simulink model "HPP"  (R2026a)
settings: Solver=ode1  StopTime=p.sim.Tstop  FixedStep=HPP_Tnet
model workspace (MAT data in the model file):
  HPP_Tnet = 0.001
  HPP_Ts = 0.001
  HPP_delays = 1
  HPP_f0 = 50
  HPP_network = 1
  HPP_simscape = 1
  buildInfo : object (value not decoded)
undefined symbols (not defined in the file): p
libraries: ee_lib x57, nesl_utility x29, fl_lib x6
(part 3 of 5)

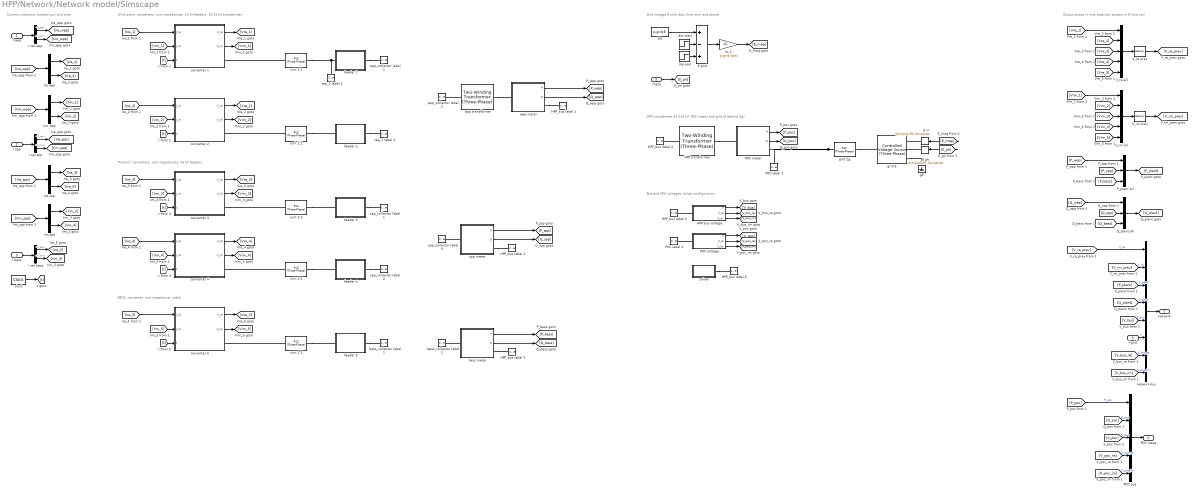
== system HPP/Network/Network model/Simscape ==
  note: Current injections (system pu) and time
  note: Wind plant: converters, unit impedances, 10 kV feeders, 10-33 kV transformer
  note: PV plant: converters, unit impedances, 33 kV feeders
  note: BESS: converter, unit impedance, cable
  note: Grid voltage E with dips (line rms) and phase
  note: HPP transformer 33-132 kV, POC meter and grid (E behind Zg)
  note: Bus and POC voltages, solver configuration
  note: Output buses (V one step old, powers in W and var)
  I wpp : Inport
  I spp : Inport  Port=2
  I bess : Inport  Port=3
  f grid : Inport  Port=4
  theta : Inport  Port=5
  E grid : Sum  Inputs=+-+
  E in : nesl_utility/Simulink-PS Converter  PhysicalDomain=network_engine_domain  SubClassName=ps_input  LeftPortType=input  RightPortType=output  PseudoPeriodic=off  Frequencies=[]  NoiseDistribution=none  NoiseParameters=[]  Unit=V  AffineConversion=off  FilteringAndDerivatives=provide  SimscapeFilterOrder=1  InputFilterTimeConstant=0.001  UdotUserProvided=0
  E ph : nesl_utility/Simulink-PS Converter  PhysicalDomain=network_engine_domain  SubClassName=ps_input  LeftPortType=input  RightPortType=output  PseudoPeriodic=off  Frequencies=[]  NoiseDistribution=none  NoiseParameters=[]  Unit=rad  AffineConversion=off  FilteringAndDerivatives=provide  SimscapeFilterOrder=1  InputFilterTimeConstant=0.001  UdotUserProvided=0
  E0 : Constant  Value=p.grid.E
  HPP bus voltage : Subsystem
  HPP transformer : ee_lib/Passive/Transformers/Two-Winding Transformer (Three-Phase)  SRated=p.net.main.S A*V  FRated=HPP_f0 Hz  Winding1Connection=ee.enum.windingconnection.Yg  VRated1=p.net.Vhpp V  Winding2Connection=ee.enum.windingconnection.Yg  VRated2=p.grid.Vpoc V  CoreType=ee.enum.coretype.threelimb  pu_Rw1=(p.net.main.uk/sqrt(1+p.net.main.XR^2))/2  pu_Rw2=(p.net.main.uk/sqrt(1+p.net.main.XR^2))/2  leakage_reactance_option=ee.enum.transformer_leakage.include  pu_Xl1=(p.net.main.uk/sqrt(1+p.net.main.XR^2))*p.net.main.XR/2  pu_Xl2=(p.net.main.uk/sqrt(1+p.net.main.XR^2))*p.net.main.XR/2  magnetizing_resistance_option=ee.enum.transformer_magnetizingResistance.include  pu_Rm=p.net.main.Rm  magnetizing_reactance_option=ee.enum.transformer_magnetizingReactance.include  saturation_option=ee.enum.transformer_saturation.exclude  pu_Xm=p.net.main.Xm  current_data=[0, .002, 1, 2]  magnetic_flux_data=[0, 1.2, 1.5, 1.51]  pu_X0=0.5  i1_specify=off  i1_priority=None  i1=[0, 0, 0] A  i1_nominal_specify=off  i1_nominal_value=1  i1_nominal_unit=A  i2_specify=off  i2_priority=None  i2=[0, 0, 0] A  i2_nominal_specify=off  i2_nominal_value=1  i2_nominal_unit=A  phi_specify=off  phi_priority=None  phi=[0, 0, 0]  phi_nominal_specify=off  phi_nominal_value=1  phi_nominal_unit=1
  HPP_bus label {1..6} (6 alike) : ConnectionLabel  Label=HPP_bus
  I sel bess : BusSelector  OutputSignals=I_re,I_im
  I sel spp : BusSelector  OutputSignals=I_re,I_im
  I sel wpp : BusSelector  OutputSignals=I_re,I_im
  Iim spp : Demux  Outputs=2
  Iim wpp : Demux  Outputs=2
  Ire spp : Demux  Outputs=2
  Ire wpp : Demux  Outputs=2
  POC bus : BusCreator  Inputs=5
  POC label 1 : ConnectionLabel  Label=POC
  POC label 2 : ConnectionLabel  Label=POC
  POC meter : Subsystem
  POC voltage : Subsystem
  P_plant all : Mux  Inputs=3
  Q_plant all : Mux  Inputs=3
  V_im all : Mux  Inputs=5
  V_im prev : Memory  InitialCondition=zeros(5,1)
  V_re all : Mux  Inputs=5
  V_re prev : Memory  InitialCondition=ones(5,1)
  bess meter : Subsystem
  bess_collector label 1 : ConnectionLabel  Label=bess_collector
  bess_collector label 2 : ConnectionLabel  Label=bess_collector
  clock : DigitalClock  SampleTime=HPP_Ts
  converter 1 : Subsystem
  converter 2 : Subsystem
  converter 3 : Subsystem
  converter 4 : Subsystem
  converter 5 : Subsystem
  dip end : Step  Time=p.grid.dip.t0 + p.grid.dip.dur  FinalValue=p.grid.dip.depth  SampleTime=0
  dip start : Step  Time=p.grid.dip.t0  FinalValue=p.grid.dip.depth  SampleTime=0
  feeder 1 : Subsystem
  feeder 2 : Subsystem
  feeder 3 : Subsystem
  feeder 4 : Subsystem
  feeder 5 : Subsystem
  gE : fl_lib/Electrical/Electrical Elements/Electrical Reference
  grid E : ee_lib/Sources/Controlled Voltage Source (Three-Phase)  input_option=ee.enum.inputType.singleFreqAC  FRated=HPP_f0 Hz
  grid Zg : ee_lib/Passive/RLC Assemblies/RLC (Three-Phase)  port_option=ee.enum.threePhasePort.composite  component_structure=ee.enum.rlc.structure.SeriesRL  R=(p.grid.Vpoc^2/(p.grid.SCR*p.grid.Pmax_poc))/sqrt(1+p.grid.XR^2) Ohm  L=(p.grid.Vpoc^2/(p.grid.SCR*p.grid.Pmax_poc))*p.grid.XR/sqrt(1+p.grid.XR^2)/(2*pi*p.grid.f0) H  C=1e-6 F  R_parasitic=0 Ohm  G_parasitic=0 1/Ohm  IL_specify=off  IL_priority=High  IL=[0, 0, 0] A  IL_nominal_specify=off  IL_nominal_value=1  IL_nominal_unit=A  VC_specify=off  VC_priority=High  VC=[0, 0, 0] V  VC_nominal_specify=off  VC_nominal_value=1  VC_nominal_unit=V
  network bus : BusCreator  Inputs=8
  solver : Subsystem  Description=Simscape solver, chosen per run by HPP_simscape (p.net.simscapeMode): Phasor (1, frequency-and-time mode, step p.sim.Ts) or EMT (2, time mode, step p.net.emtTs). See simscapeMode.  Variant=on
  spp meter : Subsystem
  spp_collector label 1 : ConnectionLabel  Label=spp_collector
  spp_collector label 2 : ConnectionLabel  Label=spp_collector
  spp_collector label 3 : ConnectionLabel  Label=spp_collector
  tap_1 label 1 : ConnectionLabel  Label=tap_1
  tap_1 label 2 : ConnectionLabel  Label=tap_1
  to V : Gain  Gain=p.grid.Vpoc
  unit Z 1 : ee_lib/Passive/RLC Assemblies/RLC (Three-Phase)  port_option=ee.enum.threePhasePort.composite  component_structure=ee.enum.rlc.structure.SeriesRL  R=(p.net.wt.unit.uk*p.net.wt.Vcol^2/(p.net.wt.unit.S*p.wt.nAgg))/sqrt(1+p.net.wt.unit.XR^2) Ohm  L=(p.net.wt.unit.uk*p.net.wt.Vcol^2/(p.net.wt.unit.S*p.wt.nAgg))*p.net.wt.unit.XR/sqrt(1+p.net.wt.unit.XR^2)/(2*pi*p.grid.f0) H  C=1e-6 F  R_parasitic=0 Ohm  G_parasitic=0 1/Ohm  IL_specify=off  IL_priority=High  IL=[0, 0, 0] A  IL_nominal_specify=off  IL_nominal_value=1  IL_nominal_unit=A  VC_specify=off  VC_priority=High  VC=[0, 0, 0] V  VC_nominal_specify=off  VC_nominal_value=1  VC_nominal_unit=V
  unit Z 2 : ee_lib/Passive/RLC Assemblies/RLC (Three-Phase)  port_option=ee.enum.threePhasePort.composite  component_structure=ee.enum.rlc.structure.SeriesRL  R=(p.net.wt.unit.uk*p.net.wt.Vcol^2/(p.net.wt.unit.S*p.wt.nAgg))/sqrt(1+p.net.wt.unit.XR^2) Ohm  L=(p.net.wt.unit.uk*p.net.wt.Vcol^2/(p.net.wt.unit.S*p.wt.nAgg))*p.net.wt.unit.XR/sqrt(1+p.net.wt.unit.XR^2)/(2*pi*p.grid.f0) H  C=1e-6 F  R_parasitic=0 Ohm  G_parasitic=0 1/Ohm  IL_specify=off  IL_priority=High  IL=[0, 0, 0] A  IL_nominal_specify=off  IL_nominal_value=1  IL_nominal_unit=A  VC_specify=off  VC_priority=High  VC=[0, 0, 0] V  VC_nominal_specify=off  VC_nominal_value=1  VC_nominal_unit=V
  unit Z 3 : ee_lib/Passive/RLC Assemblies/RLC (Three-Phase)  port_option=ee.enum.threePhasePort.composite  component_structure=ee.enum.rlc.structure.SeriesRL  R=(p.net.pv.unit.uk*p.net.pv.Vcol^2/(p.net.pv.unit.S*p.pv.nAgg))/sqrt(1+p.net.pv.unit.XR^2) Ohm  L=(p.net.pv.unit.uk*p.net.pv.Vcol^2/(p.net.pv.unit.S*p.pv.nAgg))*p.net.pv.unit.XR/sqrt(1+p.net.pv.unit.XR^2)/(2*pi*p.grid.f0) H  C=1e-6 F  R_parasitic=0 Ohm  G_parasitic=0 1/Ohm  IL_specify=off  IL_priority=High  IL=[0, 0, 0] A  IL_nominal_specify=off  IL_nominal_value=1  IL_nominal_unit=A  VC_specify=off  VC_priority=High  VC=[0, 0, 0] V  VC_nominal_specify=off  VC_nominal_value=1  VC_nominal_unit=V
  unit Z 4 : ee_lib/Passive/RLC Assemblies/RLC (Three-Phase)  port_option=ee.enum.threePhasePort.composite  component_structure=ee.enum.rlc.structure.SeriesRL  R=(p.net.pv.unit.uk*p.net.pv.Vcol^2/(p.net.pv.unit.S*p.pv.nAgg))/sqrt(1+p.net.pv.unit.XR^2) Ohm  L=(p.net.pv.unit.uk*p.net.pv.Vcol^2/(p.net.pv.unit.S*p.pv.nAgg))*p.net.pv.unit.XR/sqrt(1+p.net.pv.unit.XR^2)/(2*pi*p.grid.f0) H  C=1e-6 F  R_parasitic=0 Ohm  G_parasitic=0 1/Ohm  IL_specify=off  IL_priority=High  IL=[0, 0, 0] A  IL_nominal_specify=off  IL_nominal_value=1  IL_nominal_unit=A  VC_specify=off  VC_priority=High  VC=[0, 0, 0] V  VC_nominal_specify=off  VC_nominal_value=1  VC_nominal_unit=V
  unit Z 5 : ee_lib/Passive/RLC Assemblies/RLC (Three-Phase)  port_option=ee.enum.threePhasePort.composite  component_structure=ee.enum.rlc.structure.SeriesRL  R=(p.net.bess.unit.uk*p.net.bess.Vcol^2/(p.net.bess.unit.S*p.bess.nAgg))/sqrt(1+p.net.bess.unit.XR^2) Ohm  L=(p.net.bess.unit.uk*p.net.bess.Vcol^2/(p.net.bess.unit.S*p.bess.nAgg))*p.net.bess.unit.XR/sqrt(1+p.net.bess.unit.XR^2)/(2*pi*p.grid.f0) H  C=1e-6 F  R_parasitic=0 Ohm  G_parasitic=0 1/Ohm  IL_specify=off  IL_priority=High  IL=[0, 0, 0] A  IL_nominal_specify=off  IL_nominal_value=1  IL_nominal_unit=A  VC_specify=off  VC_priority=High  VC=[0, 0, 0] V  VC_nominal_specify=off  VC_nominal_value=1  VC_nominal_unit=V
  wpp meter : Subsystem
  wpp transformer : ee_lib/Passive/Transformers/Two-Winding Transformer (Three-Phase)  SRated=p.net.wt.plant.S A*V  FRated=HPP_f0 Hz  Winding1Connection=ee.enum.windingconnection.Yg  VRated1=p.net.wt.Vcol V  Winding2Connection=ee.enum.windingconnection.Yg  VRated2=p.net.Vhpp V  CoreType=ee.enum.coretype.threelimb  pu_Rw1=(p.net.wt.plant.uk/sqrt(1+p.net.wt.plant.XR^2))/2  pu_Rw2=(p.net.wt.plant.uk/sqrt(1+p.net.wt.plant.XR^2))/2  leakage_reactance_option=ee.enum.transformer_leakage.include  pu_Xl1=(p.net.wt.plant.uk/sqrt(1+p.net.wt.plant.XR^2))*p.net.wt.plant.XR/2  pu_Xl2=(p.net.wt.plant.uk/sqrt(1+p.net.wt.plant.XR^2))*p.net.wt.plant.XR/2  magnetizing_resistance_option=ee.enum.transformer_magnetizingResistance.include  pu_Rm=p.net.wt.plant.Rm  magnetizing_reactance_option=ee.enum.transformer_magnetizingReactance.include  saturation_option=ee.enum.transformer_saturation.exclude  pu_Xm=p.net.wt.plant.Xm  current_data=[0, .002, 1, 2]  magnetic_flux_data=[0, 1.2, 1.5, 1.51]  pu_X0=0.5  i1_specify=off  i1_priority=None  i1=[0, 0, 0] A  i1_nominal_specify=off  i1_nominal_value=1  i1_nominal_unit=A  i2_specify=off  i2_priority=None  i2=[0, 0, 0] A  i2_nominal_specify=off  i2_nominal_value=1  i2_nominal_unit=A  phi_specify=off  phi_priority=None  phi=[0, 0, 0]  phi_nominal_specify=off  phi_nominal_value=1  phi_nominal_unit=1
  wpp_collector label 1 : ConnectionLabel  Label=wpp_collector
  wpp_collector label 2 : ConnectionLabel  Label=wpp_collector
  network : Outport
  POC meas : Outport  Port=2
  wires:
  I wpp/1 -> I sel wpp/1
  I sel wpp/2 -> [Iim_wpp]  "<I_im>"
  I sel wpp/1 -> [Ire_wpp]  "<I_re>"
  [Ire_wpp] -> Ire wpp/1
  Ire wpp/2 -> [Ire_2]
  Ire wpp/1 -> [Ire_1]
  [Iim_wpp] -> Iim wpp/1
  Iim wpp/2 -> [Iim_2]
  Iim wpp/1 -> [Iim_1]
  I spp/1 -> I sel spp/1
  I sel spp/2 -> [Iim_spp]  "<I_im>"
  I sel spp/1 -> [Ire_spp]  "<I_re>"
  [Ire_spp] -> Ire spp/1
  Ire spp/2 -> [Ire_4]
  Ire spp/1 -> [Ire_3]
  [Iim_spp] -> Iim spp/1
  Iim spp/2 -> [Iim_4]
  Iim spp/1 -> [Iim_3]
  I bess/1 -> I sel bess/1
  I sel bess/2 -> [Iim_5]  "<I_im>"
  I sel bess/1 -> [Ire_5]  "<I_re>"
  clock/1 -> [t]
  [Ire_1] -> converter 1/1(I_re)
  [Iim_1] -> converter 1/2(I_im)
  [t] -> converter 1/3(t)
  converter 1/2(V_im) -> [Vim_1]
  converter 1/1(V_re) -> [Vre_1]
  [Ire_2] -> converter 2/1(I_re)
  [Iim_2] -> converter 2/2(I_im)
  [t] -> converter 2/3(t)
  converter 2/2(V_im) -> [Vim_2]
  converter 2/1(V_re) -> [Vre_2]
  wpp meter/1(P) -> [P_wpp]
  wpp meter/2(Q) -> [Q_wpp]
  [Ire_3] -> converter 3/1(I_re)
  [Iim_3] -> converter 3/2(I_im)
  [t] -> converter 3/3(t)
  converter 3/2(V_im) -> [Vim_3]
  converter 3/1(V_re) -> [Vre_3]
  [Ire_4] -> converter 4/1(I_re)
  [Iim_4] -> converter 4/2(I_im)
  [t] -> converter 4/3(t)
  converter 4/2(V_im) -> [Vim_4]
  converter 4/1(V_re) -> [Vre_4]
  spp meter/1(P) -> [P_spp]
  spp meter/2(Q) -> [Q_spp]
  [Ire_5] -> converter 5/1(I_re)
  [Iim_5] -> converter 5/2(I_im)
  [t] -> converter 5/3(t)
  converter 5/2(V_im) -> [Vim_5]
  converter 5/1(V_re) -> [Vre_5]
  bess meter/1(P) -> [P_bess]
  bess meter/2(Q) -> [Q_bess]
  E0/1 -> E grid/1
  dip start/1 -> E grid/2
  dip end/1 -> E grid/3
  E grid/1 -> to V/1
  to V/1 -> [E_mag]
  theta/1 -> [E_ph]
  [E_mag] -> E in/1
  [E_ph] -> E ph/1
  POC meter/1(P) -> [P_poc]
  POC meter/2(Q) -> [Q_poc]
  HPP bus voltage/1(V) -> [V_bus]
  HPP bus voltage/2(V_re) -> [V_bus_re]
  HPP bus voltage/3(V_im) -> [V_bus_im]
  POC voltage/1(V) -> [V_poc]
  POC voltage/2(V_re) -> [V_poc_re]
  POC voltage/3(V_im) -> [V_poc_im]
  [Vre_1] -> V_re all/1
  [Vre_2] -> V_re all/2
  [Vre_3] -> V_re all/3
  [Vre_4] -> V_re all/4
  [Vre_5] -> V_re all/5
  V_re all/1 -> V_re prev/1
  V_re prev/1 -> [V_re_prev]
  [Vim_1] -> V_im all/1
  [Vim_2] -> V_im all/2
  [Vim_3] -> V_im all/3
  [Vim_4] -> V_im all/4
  [Vim_5] -> V_im all/5
  V_im all/1 -> V_im prev/1
  V_im prev/1 -> [V_im_prev]
  [P_wpp] -> P_plant all/1
  [P_spp] -> P_plant all/2
  [P_bess] -> P_plant all/3
  P_plant all/1 -> [P_plant]
  [Q_wpp] -> Q_plant all/1
  [Q_spp] -> Q_plant all/2
  [Q_bess] -> Q_plant all/3
  Q_plant all/1 -> [Q_plant]
  [V_re_prev] -> network bus/1  "V_re"
  [V_im_prev] -> network bus/2  "V_im"
  [P_plant] -> network bus/3  "P_plant"
  [Q_plant] -> network bus/4  "Q_plant"
  [V_bus] -> network bus/5  "V_bus"
  f grid/1 -> network bus/6  "f"
  [V_bus_re] -> network bus/7  "V_bus_re"
  [V_bus_im] -> network bus/8  "V_bus_im"
  network bus/1 -> network/1
  [P_poc] -> POC bus/1  "P_poc"
  [Q_poc] -> POC bus/2  "Q_poc"
  [V_poc] -> POC bus/3  "V_poc"
  [V_poc_re] -> POC bus/4  "V_poc_re"
  [V_poc_im] -> POC bus/5  "V_poc_im"
  POC bus/1 -> POC meas/1
  connections:
  converter 1/RConn1 -- unit Z 1/LConn1
  feeder 1/LConn1 -- unit Z 1/RConn1 -- tap_1 label 1/LConn1
  feeder 1/RConn1 -- wpp_collector label 1/LConn1
  converter 2/RConn1 -- unit Z 2/LConn1
  unit Z 2/RConn1 -- feeder 2/LConn1
  feeder 2/RConn1 -- tap_1 label 2/LConn1
  wpp transformer/LConn1 -- wpp_collector label 2/LConn1
  wpp transformer/RConn1 -- wpp meter/LConn1
  wpp meter/RConn1 -- HPP_bus label 1/LConn1
  converter 3/RConn1 -- unit Z 3/LConn1
  unit Z 3/RConn1 -- feeder 3/LConn1
  feeder 3/RConn1 -- spp_collector label 1/LConn1
  converter 4/RConn1 -- unit Z 4/LConn1
  unit Z 4/RConn1 -- feeder 4/LConn1
  feeder 4/RConn1 -- spp_collector label 2/LConn1
  spp meter/LConn1 -- spp_collector label 3/LConn1
  spp meter/RConn1 -- HPP_bus label 2/LConn1
  converter 5/RConn1 -- unit Z 5/LConn1
  unit Z 5/RConn1 -- feeder 5/LConn1
  feeder 5/RConn1 -- bess_collector label 1/LConn1
  bess meter/LConn1 -- bess_collector label 2/LConn1
  bess meter/RConn1 -- HPP_bus label 3/LConn1
  HPP transformer/LConn1 -- HPP_bus label 4/LConn1
  HPP transformer/RConn1 -- POC meter/LConn1
  grid Zg/LConn1 -- POC meter/RConn1 -- POC label 1/LConn1
  grid Zg/RConn1 -- grid E/RConn1
  grid E/LConn3 -- gE/LConn1
  E in/RConn1 -- grid E/LConn1
  E ph/RConn1 -- grid E/LConn2
  HPP bus voltage/LConn1 -- HPP_bus label 5/LConn1
  POC voltage/LConn1 -- POC label 2/LConn1
  solver/RConn1 -- HPP_bus label 6/LConn1

== system HPP/PV plant/P_avail_k link/delay 3 ==
  note: 1) Add Subsystem or Model blocks as valid variant choices.
      | 2) You cannot connect blocks at this level. At simulation, connectivity is automatically
      | determined, based on the active variant and port name matching.
  u : Inport
  Fixed : Subsystem  VariantControl=HPP_delays == 1
  Variable : Subsystem  VariantControl=HPP_delays == 2
  y : Outport

== system HPP/PV plant/P_meas link/delay 3 ==
  note: 1) Add Subsystem or Model blocks as valid variant choices.
      | 2) You cannot connect blocks at this level. At simulation, connectivity is automatically
      | determined, based on the active variant and port name matching.
  u : Inport
  Fixed : Subsystem  VariantControl=HPP_delays == 1
  Variable : Subsystem  VariantControl=HPP_delays == 2
  y : Outport

== system HPP/PV plant/P_set link/delay 1 ==
  note: 1) Add Subsystem or Model blocks as valid variant choices.
      | 2) You cannot connect blocks at this level. At simulation, connectivity is automatically
      | determined, based on the active variant and port name matching.
  u : Inport
  Fixed : Subsystem  VariantControl=HPP_delays == 1
  Variable : Subsystem  VariantControl=HPP_delays == 2
  y : Outport

== system HPP/PV plant/P_set_k link/delay 1 ==
  note: 1) Add Subsystem or Model blocks as valid variant choices.
      | 2) You cannot connect blocks at this level. At simulation, connectivity is automatically
      | determined, based on the active variant and port name matching.
  u : Inport
  Fixed : Subsystem  VariantControl=HPP_delays == 1
  Variable : Subsystem  VariantControl=HPP_delays == 2
  y : Outport

== system HPP/PV plant/Q_meas link/delay 3 ==
  note: 1) Add Subsystem or Model blocks as valid variant choices.
      | 2) You cannot connect blocks at this level. At simulation, connectivity is automatically
      | determined, based on the active variant and port name matching.
  u : Inport
  Fixed : Subsystem  VariantControl=HPP_delays == 1
  Variable : Subsystem  VariantControl=HPP_delays == 2
  y : Outport

== system HPP/PV plant/Q_set link/delay 1 ==
  note: 1) Add Subsystem or Model blocks as valid variant choices.
      | 2) You cannot connect blocks at this level. At simulation, connectivity is automatically
      | determined, based on the active variant and port name matching.
  u : Inport
  Fixed : Subsystem  VariantControl=HPP_delays == 1
  Variable : Subsystem  VariantControl=HPP_delays == 2
  y : Outport

== system HPP/PV plant/Q_set_k link/delay 1 ==
  note: 1) Add Subsystem or Model blocks as valid variant choices.
      | 2) You cannot connect blocks at this level. At simulation, connectivity is automatically
      | determined, based on the active variant and port name matching.
  u : Inport
  Fixed : Subsystem  VariantControl=HPP_delays == 1
  Variable : Subsystem  VariantControl=HPP_delays == 2
  y : Outport

== system HPP/PV plant/V_meas link/delay 2 ==
  note: 1) Add Subsystem or Model blocks as valid variant choices.
      | 2) You cannot connect blocks at this level. At simulation, connectivity is automatically
      | determined, based on the active variant and port name matching.
  u : Inport
  Fixed : Subsystem  VariantControl=HPP_delays == 1
  Variable : Subsystem  VariantControl=HPP_delays == 2
  y : Outport

== system HPP/Wind plant/P_avail_k link/delay 3 ==
  note: 1) Add Subsystem or Model blocks as valid variant choices.
      | 2) You cannot connect blocks at this level. At simulation, connectivity is automatically
      | determined, based on the active variant and port name matching.
  u : Inport
  Fixed : Subsystem  VariantControl=HPP_delays == 1
  Variable : Subsystem  VariantControl=HPP_delays == 2
  y : Outport

== system HPP/Wind plant/P_meas link/delay 3 ==
  note: 1) Add Subsystem or Model blocks as valid variant choices.
      | 2) You cannot connect blocks at this level. At simulation, connectivity is automatically
      | determined, based on the active variant and port name matching.
  u : Inport
  Fixed : Subsystem  VariantControl=HPP_delays == 1
  Variable : Subsystem  VariantControl=HPP_delays == 2
  y : Outport

== system HPP/Wind plant/P_set link/delay 1 ==
  note: 1) Add Subsystem or Model blocks as valid variant choices.
      | 2) You cannot connect blocks at this level. At simulation, connectivity is automatically
      | determined, based on the active variant and port name matching.
  u : Inport
  Fixed : Subsystem  VariantControl=HPP_delays == 1
  Variable : Subsystem  VariantControl=HPP_delays == 2
  y : Outport

== system HPP/Wind plant/P_set_k link/delay 1 ==
  note: 1) Add Subsystem or Model blocks as valid variant choices.
      | 2) You cannot connect blocks at this level. At simulation, connectivity is automatically
      | determined, based on the active variant and port name matching.
  u : Inport
  Fixed : Subsystem  VariantControl=HPP_delays == 1
  Variable : Subsystem  VariantControl=HPP_delays == 2
  y : Outport

== system HPP/Wind plant/Q_meas link/delay 3 ==
  note: 1) Add Subsystem or Model blocks as valid variant choices.
      | 2) You cannot connect blocks at this level. At simulation, connectivity is automatically
      | determined, based on the active variant and port name matching.
  u : Inport
  Fixed : Subsystem  VariantControl=HPP_delays == 1
  Variable : Subsystem  VariantControl=HPP_delays == 2
  y : Outport

== system HPP/Wind plant/Q_set link/delay 1 ==
  note: 1) Add Subsystem or Model blocks as valid variant choices.
      | 2) You cannot connect blocks at this level. At simulation, connectivity is automatically
      | determined, based on the active variant and port name matching.
  u : Inport
  Fixed : Subsystem  VariantControl=HPP_delays == 1
  Variable : Subsystem  VariantControl=HPP_delays == 2
  y : Outport

== system HPP/Wind plant/Q_set_k link/delay 1 ==
  note: 1) Add Subsystem or Model blocks as valid variant choices.
      | 2) You cannot connect blocks at this level. At simulation, connectivity is automatically
      | determined, based on the active variant and port name matching.
  u : Inport
  Fixed : Subsystem  VariantControl=HPP_delays == 1
  Variable : Subsystem  VariantControl=HPP_delays == 2
  y : Outport

== system HPP/Wind plant/V_meas link/delay 2 ==
  note: 1) Add Subsystem or Model blocks as valid variant choices.
      | 2) You cannot connect blocks at this level. At simulation, connectivity is automatically
      | determined, based on the active variant and port name matching.
  u : Inport
  Fixed : Subsystem  VariantControl=HPP_delays == 1
  Variable : Subsystem  VariantControl=HPP_delays == 2
  y : Outport

== system HPP/BESS plant/P_avail_k link/delay 3/Fixed ==
  u : Inport
  Delay : Delay  DelayLength=p.comm.steps.meas_plant  InitialCondition=0  SampleTime=p.sim.Ts
  y : Outport
  wires:
  u/1 -> Delay/1
  Delay/1 -> y/1

== system HPP/BESS plant/P_avail_k link/delay 3/Variable ==
  u : Inport
  Delay : Delay  DelayLengthSource=Input port  DelayLengthUpperLimit=round(p.comm.maxDelay/p.sim.Ts)  InitialCondition=0  SampleTime=p.sim.Ts
      settings: InputPortMap=u0,p1
  steps : Constant  Value=p.comm.steps.meas_plant  OutDataTypeStr=double  SampleTime=p.sim.Ts
  y : Outport
  wires:
  u/1 -> Delay/1
  steps/1 -> Delay/2
  Delay/1 -> y/1

== system HPP/BESS plant/P_meas link/delay 3/Fixed ==
  u : Inport
  Delay : Delay  DelayLength=p.comm.steps.meas_plant  InitialCondition=0  SampleTime=p.sim.Ts
  y : Outport
  wires:
  Delay/1 -> y/1
  u/1 -> Delay/1

== system HPP/BESS plant/P_meas link/delay 3/Variable ==
  u : Inport
  Delay : Delay  DelayLengthSource=Input port  DelayLengthUpperLimit=round(p.comm.maxDelay/p.sim.Ts)  InitialCondition=0  SampleTime=p.sim.Ts
      settings: InputPortMap=u0,p1
  steps : Constant  Value=p.comm.steps.meas_plant  OutDataTypeStr=double  SampleTime=p.sim.Ts
  y : Outport
  wires:
  Delay/1 -> y/1
  steps/1 -> Delay/2
  u/1 -> Delay/1

== system HPP/BESS plant/P_set link/delay 1/Fixed ==
  u : Inport
  Delay : Delay  DelayLength=p.comm.steps.hppc_to_plant  InitialCondition=0  SampleTime=p.sim.Ts
  y : Outport
  wires:
  Delay/1 -> y/1
  u/1 -> Delay/1

== system HPP/BESS plant/P_set link/delay 1/Variable ==
  u : Inport
  Delay : Delay  DelayLengthSource=Input port  DelayLengthUpperLimit=round(p.comm.maxDelay/p.sim.Ts)  InitialCondition=0  SampleTime=p.sim.Ts
      settings: InputPortMap=u0,p1
  steps : Constant  Value=p.comm.steps.hppc_to_plant  OutDataTypeStr=double  SampleTime=p.sim.Ts
  y : Outport
  wires:
  u/1 -> Delay/1
  Delay/1 -> y/1
  steps/1 -> Delay/2

== system HPP/BESS plant/P_set_k link/delay 1/Fixed ==
  u : Inport
  Delay : Delay  DelayLength=p.comm.steps.plant_to_asset  InitialCondition=0  SampleTime=p.sim.Ts
  y : Outport
  wires:
  u/1 -> Delay/1
  Delay/1 -> y/1

== system HPP/BESS plant/P_set_k link/delay 1/Variable ==
  u : Inport
  Delay : Delay  DelayLengthSource=Input port  DelayLengthUpperLimit=round(p.comm.maxDelay/p.sim.Ts)  InitialCondition=0  SampleTime=p.sim.Ts
      settings: InputPortMap=u0,p1
  steps : Constant  Value=p.comm.steps.plant_to_asset  OutDataTypeStr=double  SampleTime=p.sim.Ts
  y : Outport
  wires:
  u/1 -> Delay/1
  steps/1 -> Delay/2
  Delay/1 -> y/1

== system HPP/BESS plant/Q_meas link/delay 3/Fixed ==
  u : Inport
  Delay : Delay  DelayLength=p.comm.steps.meas_plant  InitialCondition=0  SampleTime=p.sim.Ts
  y : Outport
  wires:
  Delay/1 -> y/1
  u/1 -> Delay/1

== system HPP/BESS plant/Q_meas link/delay 3/Variable ==
  u : Inport
  Delay : Delay  DelayLengthSource=Input port  DelayLengthUpperLimit=round(p.comm.maxDelay/p.sim.Ts)  InitialCondition=0  SampleTime=p.sim.Ts
      settings: InputPortMap=u0,p1
  steps : Constant  Value=p.comm.steps.meas_plant  OutDataTypeStr=double  SampleTime=p.sim.Ts
  y : Outport
  wires:
  u/1 -> Delay/1
  steps/1 -> Delay/2
  Delay/1 -> y/1

== system HPP/BESS plant/Q_set link/delay 1/Fixed ==
  u : Inport
  Delay : Delay  DelayLength=p.comm.steps.hppc_to_plant  InitialCondition=0  SampleTime=p.sim.Ts
  y : Outport
  wires:
  Delay/1 -> y/1
  u/1 -> Delay/1

== system HPP/BESS plant/Q_set link/delay 1/Variable ==
  u : Inport
  Delay : Delay  DelayLengthSource=Input port  DelayLengthUpperLimit=round(p.comm.maxDelay/p.sim.Ts)  InitialCondition=0  SampleTime=p.sim.Ts
      settings: InputPortMap=u0,p1
  steps : Constant  Value=p.comm.steps.hppc_to_plant  OutDataTypeStr=double  SampleTime=p.sim.Ts
  y : Outport
  wires:
  Delay/1 -> y/1
  steps/1 -> Delay/2
  u/1 -> Delay/1

== system HPP/BESS plant/Q_set_k link/delay 1/Fixed ==
  u : Inport
  Delay : Delay  DelayLength=p.comm.steps.plant_to_asset  InitialCondition=0  SampleTime=p.sim.Ts
  y : Outport
  wires:
  u/1 -> Delay/1
  Delay/1 -> y/1

== system HPP/BESS plant/Q_set_k link/delay 1/Variable ==
  u : Inport
  Delay : Delay  DelayLengthSource=Input port  DelayLengthUpperLimit=round(p.comm.maxDelay/p.sim.Ts)  InitialCondition=0  SampleTime=p.sim.Ts
      settings: InputPortMap=u0,p1
  steps : Constant  Value=p.comm.steps.plant_to_asset  OutDataTypeStr=double  SampleTime=p.sim.Ts
  y : Outport
  wires:
  steps/1 -> Delay/2
  u/1 -> Delay/1
  Delay/1 -> y/1

== system HPP/BESS plant/SOC_k link/delay 2/Fixed ==
  u : Inport
  Delay : Delay  DelayLength=p.comm.steps.meas_plant  InitialCondition=0  SampleTime=p.sim.Ts
  y : Outport
  wires:
  u/1 -> Delay/1
  Delay/1 -> y/1

== system HPP/BESS plant/SOC_k link/delay 2/Variable ==
  u : Inport
  Delay : Delay  DelayLengthSource=Input port  DelayLengthUpperLimit=round(p.comm.maxDelay/p.sim.Ts)  InitialCondition=0  SampleTime=p.sim.Ts
      settings: InputPortMap=u0,p1
  steps : Constant  Value=p.comm.steps.meas_plant  OutDataTypeStr=double  SampleTime=p.sim.Ts
  y : Outport
  wires:
  u/1 -> Delay/1
  steps/1 -> Delay/2
  Delay/1 -> y/1

== system HPP/BESS plant/V_meas link/delay 2/Fixed ==
  u : Inport
  Delay : Delay  DelayLength=p.comm.steps.meas_plant  InitialCondition=1  SampleTime=p.sim.Ts
  y : Outport
  wires:
  u/1 -> Delay/1
  Delay/1 -> y/1

== system HPP/BESS plant/V_meas link/delay 2/Variable ==
  u : Inport
  Delay : Delay  DelayLengthSource=Input port  DelayLengthUpperLimit=round(p.comm.maxDelay/p.sim.Ts)  InitialCondition=1  SampleTime=p.sim.Ts
      settings: InputPortMap=u0,p1
  steps : Constant  Value=p.comm.steps.meas_plant  OutDataTypeStr=double  SampleTime=p.sim.Ts
  y : Outport
  wires:
  u/1 -> Delay/1
  steps/1 -> Delay/2
  Delay/1 -> y/1

== system HPP/HPP controller/P_avail_spp link/delay 3/Fixed ==
  u : Inport
  Delay : Delay  DelayLength=p.comm.steps.meas_hppc  InitialCondition=0  SampleTime=p.sim.Ts
  y : Outport
  wires:
  Delay/1 -> y/1
  u/1 -> Delay/1

== system HPP/HPP controller/P_avail_spp link/delay 3/Variable ==
  u : Inport
  Delay : Delay  DelayLengthSource=Input port  DelayLengthUpperLimit=round(p.comm.maxDelay/p.sim.Ts)  InitialCondition=0  SampleTime=p.sim.Ts
      settings: InputPortMap=u0,p1
  steps : Constant  Value=p.comm.steps.meas_hppc  OutDataTypeStr=double  SampleTime=p.sim.Ts
  y : Outport
  wires:
  u/1 -> Delay/1
  steps/1 -> Delay/2
  Delay/1 -> y/1

== system HPP/HPP controller/P_avail_wpp link/delay 3/Fixed ==
  u : Inport
  Delay : Delay  DelayLength=p.comm.steps.meas_hppc  InitialCondition=0  SampleTime=p.sim.Ts
  y : Outport
  wires:
  u/1 -> Delay/1
  Delay/1 -> y/1

== system HPP/HPP controller/P_avail_wpp link/delay 3/Variable ==
  u : Inport
  Delay : Delay  DelayLengthSource=Input port  DelayLengthUpperLimit=round(p.comm.maxDelay/p.sim.Ts)  InitialCondition=0  SampleTime=p.sim.Ts
      settings: InputPortMap=u0,p1
  steps : Constant  Value=p.comm.steps.meas_hppc  OutDataTypeStr=double  SampleTime=p.sim.Ts
  y : Outport
  wires:
  u/1 -> Delay/1
  steps/1 -> Delay/2
  Delay/1 -> y/1

== system HPP/HPP controller/P_bess link/delay 3/Fixed ==
  u : Inport
  Delay : Delay  DelayLength=p.comm.steps.meas_hppc  InitialCondition=0  SampleTime=p.sim.Ts
  y : Outport
  wires:
  u/1 -> Delay/1
  Delay/1 -> y/1

== system HPP/HPP controller/P_bess link/delay 3/Variable ==
  u : Inport
  Delay : Delay  DelayLengthSource=Input port  DelayLengthUpperLimit=round(p.comm.maxDelay/p.sim.Ts)  InitialCondition=0  SampleTime=p.sim.Ts
      settings: InputPortMap=u0,p1
  steps : Constant  Value=p.comm.steps.meas_hppc  OutDataTypeStr=double  SampleTime=p.sim.Ts
  y : Outport
  wires:
  u/1 -> Delay/1
  steps/1 -> Delay/2
  Delay/1 -> y/1

== system HPP/HPP controller/P_chg_max_bess link/delay 3/Fixed ==
  u : Inport
  Delay : Delay  DelayLength=p.comm.steps.meas_hppc  InitialCondition=0  SampleTime=p.sim.Ts
  y : Outport
  wires:
  u/1 -> Delay/1
  Delay/1 -> y/1

== system HPP/HPP controller/P_chg_max_bess link/delay 3/Variable ==
  u : Inport
  Delay : Delay  DelayLengthSource=Input port  DelayLengthUpperLimit=round(p.comm.maxDelay/p.sim.Ts)  InitialCondition=0  SampleTime=p.sim.Ts
      settings: InputPortMap=u0,p1
  steps : Constant  Value=p.comm.steps.meas_hppc  OutDataTypeStr=double  SampleTime=p.sim.Ts
  y : Outport
  wires:
  u/1 -> Delay/1
  steps/1 -> Delay/2
  Delay/1 -> y/1

== system HPP/HPP controller/P_dis_max_bess link/delay 3/Fixed ==
  u : Inport
  Delay : Delay  DelayLength=p.comm.steps.meas_hppc  InitialCondition=0  SampleTime=p.sim.Ts
  y : Outport
  wires:
  u/1 -> Delay/1
  Delay/1 -> y/1

== system HPP/HPP controller/P_dis_max_bess link/delay 3/Variable ==
  u : Inport
  Delay : Delay  DelayLengthSource=Input port  DelayLengthUpperLimit=round(p.comm.maxDelay/p.sim.Ts)  InitialCondition=0  SampleTime=p.sim.Ts
      settings: InputPortMap=u0,p1
  steps : Constant  Value=p.comm.steps.meas_hppc  OutDataTypeStr=double  SampleTime=p.sim.Ts
  y : Outport
  wires:
  u/1 -> Delay/1
  steps/1 -> Delay/2
  Delay/1 -> y/1

== system HPP/HPP controller/P_poc link/delay 3/Fixed ==
  u : Inport
  Delay : Delay  DelayLength=p.comm.steps.meas_hppc  InitialCondition=0  SampleTime=p.sim.Ts
  y : Outport
  wires:
  u/1 -> Delay/1
  Delay/1 -> y/1

== system HPP/HPP controller/P_poc link/delay 3/Variable ==
  u : Inport
  Delay : Delay  DelayLengthSource=Input port  DelayLengthUpperLimit=round(p.comm.maxDelay/p.sim.Ts)  InitialCondition=0  SampleTime=p.sim.Ts
      settings: InputPortMap=u0,p1
  steps : Constant  Value=p.comm.steps.meas_hppc  OutDataTypeStr=double  SampleTime=p.sim.Ts
  y : Outport
  wires:
  u/1 -> Delay/1
  steps/1 -> Delay/2
  Delay/1 -> y/1

== system HPP/HPP controller/P_ref link/delay 2/Fixed ==
  u : Inport
  Delay : Delay  DelayLength=p.comm.steps.tso  InitialCondition=p.grid.Pref/p.ctrl.hppc.Pbase  SampleTime=p.sim.Ts
  y : Outport
  wires:
  Delay/1 -> y/1
  u/1 -> Delay/1

== system HPP/HPP controller/P_ref link/delay 2/Variable ==
  u : Inport
  Delay : Delay  DelayLengthSource=Input port  DelayLengthUpperLimit=round(p.comm.maxDelay/p.sim.Ts)  InitialCondition=p.grid.Pref/p.ctrl.hppc.Pbase  SampleTime=p.sim.Ts
      settings: InputPortMap=u0,p1
  steps : Constant  Value=p.comm.steps.tso  OutDataTypeStr=double  SampleTime=p.sim.Ts
  y : Outport
  wires:
  u/1 -> Delay/1
  steps/1 -> Delay/2
  Delay/1 -> y/1

== system HPP/HPP controller/P_spp link/delay 3/Fixed ==
  u : Inport
  Delay : Delay  DelayLength=p.comm.steps.meas_hppc  InitialCondition=0  SampleTime=p.sim.Ts
  y : Outport
  wires:
  u/1 -> Delay/1
  Delay/1 -> y/1

== system HPP/HPP controller/P_spp link/delay 3/Variable ==
  u : Inport
  Delay : Delay  DelayLengthSource=Input port  DelayLengthUpperLimit=round(p.comm.maxDelay/p.sim.Ts)  InitialCondition=0  SampleTime=p.sim.Ts
      settings: InputPortMap=u0,p1
  steps : Constant  Value=p.comm.steps.meas_hppc  OutDataTypeStr=double  SampleTime=p.sim.Ts
  y : Outport
  wires:
  u/1 -> Delay/1
  steps/1 -> Delay/2
  Delay/1 -> y/1

== system HPP/HPP controller/P_wpp link/delay 3/Fixed ==
  u : Inport
  Delay : Delay  DelayLength=p.comm.steps.meas_hppc  InitialCondition=0  SampleTime=p.sim.Ts
  y : Outport
  wires:
  u/1 -> Delay/1
  Delay/1 -> y/1

== system HPP/HPP controller/P_wpp link/delay 3/Variable ==
  u : Inport
  Delay : Delay  DelayLengthSource=Input port  DelayLengthUpperLimit=round(p.comm.maxDelay/p.sim.Ts)  InitialCondition=0  SampleTime=p.sim.Ts
      settings: InputPortMap=u0,p1
  steps : Constant  Value=p.comm.steps.meas_hppc  OutDataTypeStr=double  SampleTime=p.sim.Ts
  y : Outport
  wires:
  u/1 -> Delay/1
  steps/1 -> Delay/2
  Delay/1 -> y/1

== system HPP/HPP controller/Q_bess link/delay 3/Fixed ==
  u : Inport
  Delay : Delay  DelayLength=p.comm.steps.meas_hppc  InitialCondition=0  SampleTime=p.sim.Ts
  y : Outport
  wires:
  u/1 -> Delay/1
  Delay/1 -> y/1

== system HPP/HPP controller/Q_bess link/delay 3/Variable ==
  u : Inport
  Delay : Delay  DelayLengthSource=Input port  DelayLengthUpperLimit=round(p.comm.maxDelay/p.sim.Ts)  InitialCondition=0  SampleTime=p.sim.Ts
      settings: InputPortMap=u0,p1
  steps : Constant  Value=p.comm.steps.meas_hppc  OutDataTypeStr=double  SampleTime=p.sim.Ts
  y : Outport
  wires:
  u/1 -> Delay/1
  steps/1 -> Delay/2
  Delay/1 -> y/1

== system HPP/HPP controller/Q_poc link/delay 3/Fixed ==
  u : Inport
  Delay : Delay  DelayLength=p.comm.steps.meas_hppc  InitialCondition=0  SampleTime=p.sim.Ts
  y : Outport
  wires:
  u/1 -> Delay/1
  Delay/1 -> y/1

== system HPP/HPP controller/Q_poc link/delay 3/Variable ==
  u : Inport
  Delay : Delay  DelayLengthSource=Input port  DelayLengthUpperLimit=round(p.comm.maxDelay/p.sim.Ts)  InitialCondition=0  SampleTime=p.sim.Ts
      settings: InputPortMap=u0,p1
  steps : Constant  Value=p.comm.steps.meas_hppc  OutDataTypeStr=double  SampleTime=p.sim.Ts
  y : Outport
  wires:
  u/1 -> Delay/1
  steps/1 -> Delay/2
  Delay/1 -> y/1

== system HPP/HPP controller/Q_ref link/delay 2/Fixed ==
  u : Inport
  Delay : Delay  DelayLength=p.comm.steps.tso  InitialCondition=p.grid.Qref/p.ctrl.hppc.Pbase  SampleTime=p.sim.Ts
  y : Outport
  wires:
  u/1 -> Delay/1
  Delay/1 -> y/1

== system HPP/HPP controller/Q_ref link/delay 2/Variable ==
  u : Inport
  Delay : Delay  DelayLengthSource=Input port  DelayLengthUpperLimit=round(p.comm.maxDelay/p.sim.Ts)  InitialCondition=p.grid.Qref/p.ctrl.hppc.Pbase  SampleTime=p.sim.Ts
      settings: InputPortMap=u0,p1
  steps : Constant  Value=p.comm.steps.tso  OutDataTypeStr=double  SampleTime=p.sim.Ts
  y : Outport
  wires:
  u/1 -> Delay/1
  steps/1 -> Delay/2
  Delay/1 -> y/1

== system HPP/HPP controller/Q_sat_bess link/delay 2/Fixed ==
  u : Inport
  Delay : Delay  DelayLength=p.comm.steps.meas_hppc  InitialCondition=0  SampleTime=p.sim.Ts
  y : Outport
  wires:
  u/1 -> Delay/1
  Delay/1 -> y/1

== system HPP/HPP controller/Q_sat_bess link/delay 2/Variable ==
  u : Inport
  Delay : Delay  DelayLengthSource=Input port  DelayLengthUpperLimit=round(p.comm.maxDelay/p.sim.Ts)  InitialCondition=0  SampleTime=p.sim.Ts
      settings: InputPortMap=u0,p1
  steps : Constant  Value=p.comm.steps.meas_hppc  OutDataTypeStr=double  SampleTime=p.sim.Ts
  y : Outport
  wires:
  u/1 -> Delay/1
  steps/1 -> Delay/2
  Delay/1 -> y/1

== system HPP/HPP controller/Q_sat_spp link/delay 2/Fixed ==
  u : Inport
  Delay : Delay  DelayLength=p.comm.steps.meas_hppc  InitialCondition=0  SampleTime=p.sim.Ts
  y : Outport
  wires:
  u/1 -> Delay/1
  Delay/1 -> y/1

== system HPP/HPP controller/Q_sat_spp link/delay 2/Variable ==
  u : Inport
  Delay : Delay  DelayLengthSource=Input port  DelayLengthUpperLimit=round(p.comm.maxDelay/p.sim.Ts)  InitialCondition=0  SampleTime=p.sim.Ts
      settings: InputPortMap=u0,p1
  steps : Constant  Value=p.comm.steps.meas_hppc  OutDataTypeStr=double  SampleTime=p.sim.Ts
  y : Outport
  wires:
  u/1 -> Delay/1
  steps/1 -> Delay/2
  Delay/1 -> y/1

== system HPP/HPP controller/Q_sat_wpp link/delay 2/Fixed ==
  u : Inport
  Delay : Delay  DelayLength=p.comm.steps.meas_hppc  InitialCondition=0  SampleTime=p.sim.Ts
  y : Outport
  wires:
  u/1 -> Delay/1
  Delay/1 -> y/1

== system HPP/HPP controller/Q_sat_wpp link/delay 2/Variable ==
  u : Inport
  Delay : Delay  DelayLengthSource=Input port  DelayLengthUpperLimit=round(p.comm.maxDelay/p.sim.Ts)  InitialCondition=0  SampleTime=p.sim.Ts
      settings: InputPortMap=u0,p1
  steps : Constant  Value=p.comm.steps.meas_hppc  OutDataTypeStr=double  SampleTime=p.sim.Ts
  y : Outport
  wires:
  u/1 -> Delay/1
  steps/1 -> Delay/2
  Delay/1 -> y/1

== system HPP/HPP controller/Q_spp link/delay 3/Fixed ==
  u : Inport
  Delay : Delay  DelayLength=p.comm.steps.meas_hppc  InitialCondition=0  SampleTime=p.sim.Ts
  y : Outport
  wires:
  u/1 -> Delay/1
  Delay/1 -> y/1

== system HPP/HPP controller/Q_spp link/delay 3/Variable ==
  u : Inport
  Delay : Delay  DelayLengthSource=Input port  DelayLengthUpperLimit=round(p.comm.maxDelay/p.sim.Ts)  InitialCondition=0  SampleTime=p.sim.Ts
      settings: InputPortMap=u0,p1
  steps : Constant  Value=p.comm.steps.meas_hppc  OutDataTypeStr=double  SampleTime=p.sim.Ts
  y : Outport
  wires:
  u/1 -> Delay/1
  steps/1 -> Delay/2
  Delay/1 -> y/1

== system HPP/HPP controller/Q_wpp link/delay 3/Fixed ==
  u : Inport
  Delay : Delay  DelayLength=p.comm.steps.meas_hppc  InitialCondition=0  SampleTime=p.sim.Ts
  y : Outport
  wires:
  u/1 -> Delay/1
  Delay/1 -> y/1

== system HPP/HPP controller/Q_wpp link/delay 3/Variable ==
  u : Inport
  Delay : Delay  DelayLengthSource=Input port  DelayLengthUpperLimit=round(p.comm.maxDelay/p.sim.Ts)  InitialCondition=0  SampleTime=p.sim.Ts
      settings: InputPortMap=u0,p1
  steps : Constant  Value=p.comm.steps.meas_hppc  OutDataTypeStr=double  SampleTime=p.sim.Ts
  y : Outport
  wires:
  u/1 -> Delay/1
  steps/1 -> Delay/2
  Delay/1 -> y/1

== system HPP/HPP controller/SOC_bess link/delay 2/Fixed ==
  u : Inport
  Delay : Delay  DelayLength=p.comm.steps.meas_hppc  InitialCondition=0  SampleTime=p.sim.Ts
  y : Outport
  wires:
  u/1 -> Delay/1
  Delay/1 -> y/1

== system HPP/HPP controller/SOC_bess link/delay 2/Variable ==
  u : Inport
  Delay : Delay  DelayLengthSource=Input port  DelayLengthUpperLimit=round(p.comm.maxDelay/p.sim.Ts)  InitialCondition=0  SampleTime=p.sim.Ts
      settings: InputPortMap=u0,p1
  steps : Constant  Value=p.comm.steps.meas_hppc  OutDataTypeStr=double  SampleTime=p.sim.Ts
  y : Outport
  wires:
  u/1 -> Delay/1
  steps/1 -> Delay/2
  Delay/1 -> y/1

== system HPP/HPP controller/V_poc link/delay 2/Fixed ==
  u : Inport
  Delay : Delay  DelayLength=p.comm.steps.meas_hppc  InitialCondition=1  SampleTime=p.sim.Ts
  y : Outport
  wires:
  u/1 -> Delay/1
  Delay/1 -> y/1

== system HPP/HPP controller/V_poc link/delay 2/Variable ==
  u : Inport
  Delay : Delay  DelayLengthSource=Input port  DelayLengthUpperLimit=round(p.comm.maxDelay/p.sim.Ts)  InitialCondition=1  SampleTime=p.sim.Ts
      settings: InputPortMap=u0,p1
  steps : Constant  Value=p.comm.steps.meas_hppc  OutDataTypeStr=double  SampleTime=p.sim.Ts
  y : Outport
  wires:
  u/1 -> Delay/1
  steps/1 -> Delay/2
  Delay/1 -> y/1

== system HPP/Network/Grid frequency/swing equation/Pm state ==
  dx : Inport
  active : Inport  Port=2
  Ts : Gain  Gain=p.sim.Ts
  active? : Switch  Criteria=u2 ~= 0  SaturateOnIntegerOverflow=off  InputSameDT=off
  x[k-1] : UnitDelay  SampleTime=-1
  x[k-1] + Ts dx : Sum
  x : Outport
  x_prev : Outport  Port=2
  wires:
  dx/1 -> Ts/1
  x[k-1]/1 -> x[k-1] + Ts dx/1, active?/3, x_prev/1  "x[k-1]"
  Ts/1 -> x[k-1] + Ts dx/2
  x[k-1] + Ts dx/1 -> active?/1
  active/1 -> active?/2
  active?/1 -> x/1, x[k-1]/1  "x"

== system HPP/Network/Grid frequency/swing equation/w state ==
  dx : Inport
  active : Inport  Port=2
  Ts : Gain  Gain=p.sim.Ts
  active? : Switch  Criteria=u2 ~= 0  SaturateOnIntegerOverflow=off  InputSameDT=off
  x[k-1] : UnitDelay  SampleTime=-1
  x[k-1] + Ts dx : Sum
  x : Outport
  x_prev : Outport  Port=2
  wires:
  dx/1 -> Ts/1
  x[k-1]/1 -> x[k-1] + Ts dx/1, active?/3, x_prev/1  "x[k-1]"
  Ts/1 -> x[k-1] + Ts dx/2
  x[k-1] + Ts dx/1 -> active?/1
  active/1 -> active?/2
  active?/1 -> x/1, x[k-1]/1  "x"

== system HPP/Network/Grid frequency/swing equation/xg state ==
  dx : Inport
  active : Inport  Port=2
  Ts : Gain  Gain=p.sim.Ts
  active? : Switch  Criteria=u2 ~= 0  SaturateOnIntegerOverflow=off  InputSameDT=off
  x[k-1] : UnitDelay  SampleTime=-1
  x[k-1] + Ts dx : Sum
  x : Outport
  x_prev : Outport  Port=2
  wires:
  dx/1 -> Ts/1
  x[k-1]/1 -> x[k-1] + Ts dx/1, active?/3, x_prev/1  "x[k-1]"
  Ts/1 -> x[k-1] + Ts dx/2
  x[k-1] + Ts dx/1 -> active?/1
  active/1 -> active?/2
  active?/1 -> x/1, x[k-1]/1  "x"

== system HPP/Network/Network model/Simscape/HPP bus voltage ==
  Vs : ee_lib/Sensors & Transducers/Phase Voltage Sensor (Three-Phase)  port_option=ee.enum.threePhasePort.composite
  abs : Math  Operator=hypot
  clock : DigitalClock  SampleTime=HPP_Ts
  gn : ee_lib/Connectors & References/Grounded Neutral (Three-Phase)  port_option=ee.enum.threePhasePort.composite
  phasor : Subsystem
  v : nesl_utility/PS-Simulink Converter  PhysicalDomain=network_engine_domain  SubClassName=ps_output  LeftPortType=input  RightPortType=output  PseudoPeriodic=off  Frequencies=[]  VectorFormat=inherit  Unit=inherit  AffineConversion=off
  a : PMIOPort  Side=Left
  V : Outport
  V_re : Outport  Port=2
  V_im : Outport  Port=3
  wires:
  v/1 -> phasor/1(v)
  clock/1 -> phasor/2(t)
  phasor/1(V_re) -> abs/1, V_re/1
  phasor/2(V_im) -> abs/2, V_im/1
  abs/1 -> V/1
  connections:
  a/RConn1 -- Vs/LConn1
  Vs/RConn2 -- gn/LConn1
  Vs/RConn1 -- v/LConn1

== system HPP/Network/Network model/Simscape/POC meter ==
  P hold : ZeroOrderHold  SampleTime=HPP_Ts
  P out : nesl_utility/PS-Simulink Converter  PhysicalDomain=network_engine_domain  SubClassName=ps_output  LeftPortType=input  RightPortType=output  PseudoPeriodic=off  Frequencies=[]  VectorFormat=inherit  Unit=inherit  AffineConversion=off
  PQ : ee_lib/Sensors & Transducers/Power Sensor (Three-Phase)  port_option=ee.enum.threePhasePort.composite  load_type=ee.enum.passive.type_balanced.balanced  f0=HPP_f0 Hz
  Q hold : ZeroOrderHold  SampleTime=HPP_Ts
  Q out : nesl_utility/PS-Simulink Converter  PhysicalDomain=network_engine_domain  SubClassName=ps_output  LeftPortType=input  RightPortType=output  PseudoPeriodic=off  Frequencies=[]  VectorFormat=inherit  Unit=inherit  AffineConversion=off
  a : PMIOPort  Side=Left
  b : PMIOPort  Port=2  Side=Right
  P : Outport
  Q : Outport  Port=2
  wires:
  P out/1 -> P hold/1
  P hold/1 -> P/1
  Q out/1 -> Q hold/1
  Q hold/1 -> Q/1
  connections:
  a/RConn1 -- PQ/LConn1
  b/RConn1 -- PQ/RConn1
  PQ/LConn2 -- P out/LConn1
  PQ/LConn3 -- Q out/LConn1

== system HPP/Network/Network model/Simscape/POC voltage ==
  Vs : ee_lib/Sensors & Transducers/Phase Voltage Sensor (Three-Phase)  port_option=ee.enum.threePhasePort.composite
  abs : Math  Operator=hypot
  clock : DigitalClock  SampleTime=HPP_Ts
  gn : ee_lib/Connectors & References/Grounded Neutral (Three-Phase)  port_option=ee.enum.threePhasePort.composite
  phasor : Subsystem
  v : nesl_utility/PS-Simulink Converter  PhysicalDomain=network_engine_domain  SubClassName=ps_output  LeftPortType=input  RightPortType=output  PseudoPeriodic=off  Frequencies=[]  VectorFormat=inherit  Unit=inherit  AffineConversion=off
  a : PMIOPort  Side=Left
  V : Outport
  V_re : Outport  Port=2
  V_im : Outport  Port=3
  wires:
  v/1 -> phasor/1(v)
  clock/1 -> phasor/2(t)
  phasor/1(V_re) -> abs/1, V_re/1
  phasor/2(V_im) -> abs/2, V_im/1
  abs/1 -> V/1
  connections:
  a/RConn1 -- Vs/LConn1
  Vs/RConn2 -- gn/LConn1
  Vs/RConn1 -- v/LConn1

== system HPP/Network/Network model/Simscape/bess meter ==
  P hold : ZeroOrderHold  SampleTime=HPP_Ts
  P out : nesl_utility/PS-Simulink Converter  PhysicalDomain=network_engine_domain  SubClassName=ps_output  LeftPortType=input  RightPortType=output  PseudoPeriodic=off  Frequencies=[]  VectorFormat=inherit  Unit=inherit  AffineConversion=off
  PQ : ee_lib/Sensors & Transducers/Power Sensor (Three-Phase)  port_option=ee.enum.threePhasePort.composite  load_type=ee.enum.passive.type_balanced.balanced  f0=HPP_f0 Hz
  Q hold : ZeroOrderHold  SampleTime=HPP_Ts
  Q out : nesl_utility/PS-Simulink Converter  PhysicalDomain=network_engine_domain  SubClassName=ps_output  LeftPortType=input  RightPortType=output  PseudoPeriodic=off  Frequencies=[]  VectorFormat=inherit  Unit=inherit  AffineConversion=off
  a : PMIOPort  Side=Left
  b : PMIOPort  Port=2  Side=Right
  P : Outport
  Q : Outport  Port=2
  wires:
  P out/1 -> P hold/1
  P hold/1 -> P/1
  Q out/1 -> Q hold/1
  Q hold/1 -> Q/1
  connections:
  a/RConn1 -- PQ/LConn1
  b/RConn1 -- PQ/RConn1
  PQ/LConn2 -- P out/LConn1
  PQ/LConn3 -- Q out/LConn1

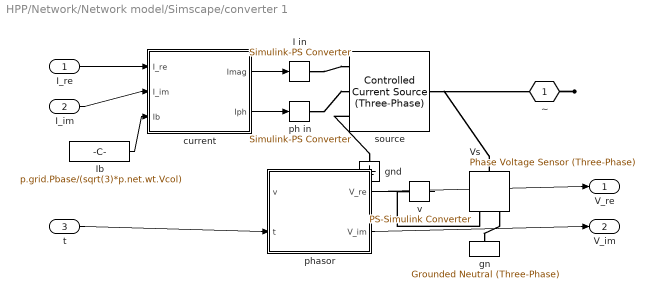
== system HPP/Network/Network model/Simscape/converter 1 ==
  I_re : Inport
  I_im : Inport  Port=2
  t : Inport  Port=3
  I in : nesl_utility/Simulink-PS Converter  PhysicalDomain=network_engine_domain  SubClassName=ps_input  LeftPortType=input  RightPortType=output  PseudoPeriodic=off  Frequencies=[]  NoiseDistribution=none  NoiseParameters=[]  Unit=A  AffineConversion=off  FilteringAndDerivatives=provide  SimscapeFilterOrder=1  InputFilterTimeConstant=0.001  UdotUserProvided=0
  Ib : Constant  Value=p.grid.Pbase/(sqrt(3)*p.net.wt.Vcol)
  Vs : ee_lib/Sensors & Transducers/Phase Voltage Sensor (Three-Phase)  port_option=ee.enum.threePhasePort.composite
  current : MATLAB Function  TreatAsAtomicUnit=on
  gn : ee_lib/Connectors & References/Grounded Neutral (Three-Phase)  port_option=ee.enum.threePhasePort.composite
  gnd : fl_lib/Electrical/Electrical Elements/Electrical Reference
  ph in : nesl_utility/Simulink-PS Converter  PhysicalDomain=network_engine_domain  SubClassName=ps_input  LeftPortType=input  RightPortType=output  PseudoPeriodic=off  Frequencies=[]  NoiseDistribution=none  NoiseParameters=[]  Unit=rad  AffineConversion=off  FilteringAndDerivatives=provide  SimscapeFilterOrder=1  InputFilterTimeConstant=0.001  UdotUserProvided=0
  phasor : Subsystem
  source : ee_lib/Sources/Controlled Current Source (Three-Phase)  port_option=ee.enum.threePhasePort.composite  input_option=ee.enum.inputType.singleFreqAC  FRated=HPP_f0 Hz  G_parasitic=0 1/Ohm
  v : nesl_utility/PS-Simulink Converter  PhysicalDomain=network_engine_domain  SubClassName=ps_output  LeftPortType=input  RightPortType=output  PseudoPeriodic=off  Frequencies=[]  VectorFormat=inherit  Unit=inherit  AffineConversion=off
  ~ : PMIOPort  Side=Right
  V_re : Outport
  V_im : Outport  Port=2
  wires:
  I_re/1 -> current/1(I_re)
  I_im/1 -> current/2(I_im)
  Ib/1 -> current/3(Ib)
  current/1(Imag) -> I in/1
  current/2(Iph) -> ph in/1
  v/1 -> phasor/1(v)
  t/1 -> phasor/2(t)
  phasor/1(V_re) -> V_re/1
  phasor/2(V_im) -> V_im/1
  connections:
  I in/RConn1 -- source/LConn1
  ph in/RConn1 -- source/LConn2
  source/LConn3 -- gnd/LConn1
  ~/RConn1 -- source/RConn1 -- Vs/LConn1
  Vs/RConn2 -- gn/LConn1
  Vs/RConn1 -- v/LConn1
